simulink model "KINvasion"  (Simulink 7.5)
settings: Solver=ode4  SolverMode=SingleTasking  StartTime=0.0  StopTime=inf  FixedStep=0.0005  RelTol=1e-3
StartFcn:
  |  warndlg('Dexterit-E models cannot run under simulation. Please compile your model and run it from within Dexterit-E.');set_param(gcs,'SimulationCommand','stop')
undefined symbols (not defined in the file or in its folder): Process_Video_CMD, Video
libraries: xpclib x5, General x3, KINARM_general x1, KINARM_EP_loads x1
(part 2 of 3)

== stateflow chart Trial_Control ==
  settings: sampleTime=0.001
  state Initialize/
    // Initialize all variables at the start of the game
    logging_enable = 0;
    game_state=0;
    InitializeAll();
    NullVCODES();
    Continue=1;
  state Main_Trial/
    state GameOn/
      // Set up a level and run the game
      logging_enable=1;
      EnemyNum=Trial_Protocol[EnemyNumber];
      Difficulty=Trial_Protocol[DifficultyNumber];
      MoneyNum=Trial_Protocol[MoneyDrops];
      BossNum=Trial_Protocol[BossNumber];
      GameLoop(1);
      during:
      GameLoop(0);
      exit:
      TitleText();
      ZeroForce();
    state Win/
      // The player won.
      // Continue to interstate
    state Loss/
      // The player lost
      // Set variable to skip
      // all futher levels
      Continue=0;
    state Store/
      // Show the store to the player
      game_state=0;
      ZeroForce();
      Level=Level+1;
      during:
      StoreLoop();
    GameOn -> Win [order 2] : [game_state==2]
    GameOn -> Loss [order 1] : [game_state==3]
    Store -> GameOn : [game_state==1 || TWP[DemoMode]!=0]
  state Inter_Trial_State/
    tickCount=10;
    logging_enable = 0;
    e_Trial_End;
  state Continuing/
    // Does the player get
    // to play another
    // level or did they
    // lose?
  Main_Trial -> Inter_Trial_State : e_ExitTrialNow/
      | // if e_ExitTrialNow event occurs,
      | tickCount=1;
  Initialize -> Store
  (default) -> Initialize
  Win -> Inter_Trial_State : after(2000, e_clk)
  Inter_Trial_State -> Continuing : after(tickCount, e_clk)
  Loss -> Inter_Trial_State : after(10000, e_clk)
  Continuing -> Store [order 1] : [Continue==1]
  Continuing -> Inter_Trial_State [order 2] : [Continue==0]
  data: Initialize function_input double; RRRGGGBBB function_input double; RRGGBBAA function_output uint32; out function_output double size=[1 2]; in function_input double; out function_output double size=[1 3]; in function_input double; logging_enable output double; Trial_Protocol input double; tickCount local double; EnemyNum local double; Difficulty local double; game_state local double; Forces output double size=[1 4]; Continue local double; Money local double; Score local double; VCODES output double size=[100,70]; Upgrades local double size=5; TWP input double; KINARMdata input double; ForcePlatedata input double; seed input double; Level local double; MoneyNum local double; BossNum local double
  events: e_clk input RISING_EDGE_EVENT; e_ExitTrialNow input EITHER_EDGE_EVENT; e_Trial_End output EITHER_EDGE_EVENT
  function StoreLoop:
    | function StoreLoop
    | % This function shows and regulates the game's behaviour while the player
    | % is buying and selling upgrades.
    | %
    | % Upgrades is a 1x5 vector that tracks how many of each upgrade the player
    | % has purchased.
    | %
    | 
    |     persistent SelectTimer; % Used to limit time between purchases
    |     
    |     Forces=zeros(1,4); % Don't need forces here
    |     
    |     if isempty(SelectTimer)
    |         SelectTimer=0;
    |     end
    |     
    |     VCODES=zeros(100,70);
    |     
    |     % increments of vertical space for display
    |     increment=(TWP(WindowMaxY)-TWP(WindowMinY))/8; 
    |     
    |     for i=1:2
    |         if i==1
    |             active_arm=KINARMdata(3,1);			%choose dominant arm first
    |         else
    |             active_arm=3-KINARMdata(3,1);		%choose non-dominant arm 2nd
    |         end
    |         
    |         VCODES(i,1)=1;							%target_type of circle
    |         VCODES(i,2)=1;                          %show target
    |         VCODES(i,5)=colourshift(100255);        %fill colour
    |         VCODES(i,6)=colourshift(100255);		%stroke colour
    |         VCODES(i,7)=0;							%no stroke width
    |         VCODES(i,9)=100;                        %100% opacity
    |         VCODES(i,10)=0.005;                     %radius (m)
    |         feedfwd=KINARMdata(3,2);
    |         VCODES(i,3)=KINARMdata(active_arm,23) + KINARMdata(active_arm,25)*feedfwd;
    |         VCODES(i,4)=KINARMdata(active_arm,24) + KINARMdata(active_arm,26)*feedfwd;
    |         
    |         if SelectTimer==0
    |             % If using the right hand, buy things
    |             if ((sum(KINARMdata(active_arm,47:48).^2)>TWP(FireTorque)^2)&& i==1)
    |                 SelectTimer=600;
    |                 if (IsOver(VCODES(i,4))==2 && Money>=10)
    |                     Money=Money-10;
    |                     Upgrades(1)=Upgrades(1)+1;
    |                 elseif (IsOver(VCODES(i,4))==3 && Money>=15)
    |                     Money=Money-15;
    |                     Upgrades(2)=Upgrades(2)+1;
    |                 elseif (IsOver(VCODES(i,4))==4 && Money>=25)
    |                     Money=Money-25;
    |                     Upgrades(4)=Upgrades(4)+1;
    |                 elseif (IsOver(VCODES(i,4))==5 && Money>=50)
    |                     Money=Money-50;
    |                     Upgrades(3)=Upgrades(3)+1;
    |                 elseif IsOver(VCODES(i,4))==7
    |                     game_state=1;
    |                 end
    |                     
    |             % If using the left hand, sell things
    |             elseif ((sum(KINARMdata(active_arm,47:48).^2)>TWP(FireTorque)^2)&& i==2)
    |                 SelectTimer=600;
    |                 if (IsOver(VCODES(i,4))==2 && Upgrades(1)>=1)
    |                     Money=Money+10;
    |                     Upgrades(1)=Upgrades(1)-1;
    |                 elseif (IsOver(VCODES(i,4))==3 && Upgrades(2)>=1)
    |                     Money=Money+15;
    |                     Upgrades(2)=Upgrades(2)-1;
    |                 elseif (IsOver(VCODES(i,4))==4 && Upgrades(4)>=1)
    |                     Money=Money+25;
    |                     Upgrades(4)=Upgrades(4)-1;
    |                 elseif (IsOver(VCODES(i,4))==5 && Upgrades(3)>=1)
    |                     Money=Money+50;
    |                     Upgrades(3)=Upgrades(3)-1;
    |                 elseif IsOver(VCODES(i,4))==7
    |                     game_state=1;
    |                 end
    |             end
    |         else
    |             SelectTimer=SelectTimer-1;
    |         end
    |         
    |     end
    |     
    |     % Show score and money
    |     VCODES(3,:)=titleCode(...
    |         ['SCORE ',numberText3(Score),' $',numberText3(Money)],...
    |         [TWP(WindowMaxX),TWP(WindowMaxY)],0.05);
    |     
    |     % Show buying options
    |     VCODES(4,:)=titleCode(['Shields          $10 / ',(48+floor(Upgrades(1)/10)), 48+mod(Upgrades(1),10)],...
    |         [(TWP(WindowMaxX)+TWP(WindowMinX))/2,(TWP(WindowMaxY)-increment*2)],0.04);
    |     VCODES(5,:)=titleCode(['Charge Rate     $15 / ',(48+floor(Upgrades(2)/10)), 48+mod(Upgrades(2),10)],...
    |         [(TWP(WindowMaxX)+TWP(WindowMinX))/2,(TWP(WindowMaxY)-increment*3)],0.04);
    |     VCODES(6,:)=titleCode(['Bombs          $25 / ',(48+floor(Upgrades(4)/10)), 48+mod(Upgrades(4),10)],...
    |         [(TWP(WindowMaxX)+TWP(WindowMinX))/2,(TWP(WindowMaxY)-increment*4)],0.04);
    |     VCODES(7,:)=titleCode(['AutoCannon  $50 / ',(48+floor(Upgrades(3)/10)), 48+mod(Upgrades(3),10)],...
    |         [(TWP(WindowMaxX)+TWP(WindowMinX))/2,(TWP(WindowMaxY)-increment*5)],0.04);
    |     
    |     % Show option to continue to the play stage
    |     VCODES(8,:)=titleCode('DONE',...
    |         [(TWP(WindowMaxX)+TWP(WindowMinX))/2,(TWP(WindowMaxY)-increment*7)],0.04);
    | 
    | end
    | 
    | %%%%%%%%%%%%%  ADDITIONAL FUNCTIONS %%%%%%%%%%%%%%%
    | 
    | function VC = titleCode(str,loc,size)
    | % This function creates a VCODE with some text at a certain
    | % size and global location.
    | 
    |     VC=zeros(1,70);
    |     VC(1,1)=11;                             %target_type of labelled circle
    |     VC(1,2)=1;                              %show target
    |     VC(1,3) = loc(1);
    |     VC(1,4) = loc(2);
    |     VC(1,5)=colourshift(255);               %fill colour
    |     VC(1,6)=colourshift(255);               %stroke colour
    |     VC(1,7)=0.00;                           %no stroke width
    |     VC(1,9)=100;                            %100% opacity
    |     VC(1,10)=0.0;                           %radius (m)
    |     VC(1,15:(length(str)+14))=uint16(str);  %str in letters
    |     VC(1,65)=colourshift(254254254);        %text color
    |     VC(1,66)=size;                          %text height (m)
    |     
    | end
    | 
    | function inc=IsOver(locy)
    | % This function finds the increment of vertical space that the location
    | % is in. To allow for discrimination of choices
    | 
    |     inc=TWP(WindowMaxY)-locy;
    |     inc=inc/((TWP(WindowMaxY)-TWP(WindowMinY))/8);
    |     inc=floor(inc+0.5);
    | 
    | end
  function GameLoop(Initialize):
    | function GameLoop(Initialize)
    | % This function is iterated every millisecond of game time. It shows all
    | % the graphics by creating VCODEs, and updates the location and state of
    | % all game elements.
    | 
    |     % Some persistent variables that are needed between game loop iterations
    |     persistent Power Health Shields Enemies Bosses Shots firstrun startcounter forcedata Bombs Moneys;
    |     
    |     MaxShips=50;
    |     MaxShots=70;
    |     MaxMoneys=50;
    |     MaxBosses=15;
    |     
    |     % Instantiate random seed.
    |     if isempty(firstrun)
    |         rand('twister',seed);
    |         firstrun=1;
    |     end
    | 
    |     Forces=zeros(1,4);
    |     T=[0,0];
    |     temp=0;
    |     
    |     VCODES=zeros(100,70);
    |     
    |     if (isempty(forcedata) || Initialize==1)
    |         forcedata=[ForcePlatedata(10),ForcePlatedata(3),0,0];
    |     end
    |     forcedata(3:4)=abs([ForcePlatedata(10),ForcePlatedata(3)]-forcedata(1:2));
    |     forcedata(1:2)=[ForcePlatedata(10),ForcePlatedata(3)];
    |     
    |     if (isempty(Bombs) || Initialize==1)
    |         Bombs=[0,0,0,0,0,0];
    |     end
    |     
    |     
    |     if (isempty(Power) || Initialize==1)
    |         Power=[100,100,100];
    |     end
    |     
    |     if (isempty(Health) || Initialize==1)
    |         Health=0;
    |     end
    |     
    |      if (isempty(Shields) || Initialize==1)
    |         Shields=0;
    |     end
    |     
    |     if (isempty(startcounter) || Initialize==1)
    |         startcounter=1;
    |     end
    |     
    |     if (isempty(Shots) || Initialize==1)
    |         Shots=zeros(MaxShots,6);
    |     end
    |     
    |     if isempty(Enemies)
    |         Enemies=zeros(MaxShips,9);
    |     end
    |     
    |     if isempty(Bosses)
    |         Bosses=zeros(MaxBosses,9);
    |     end
    |     
    |     if isempty(Moneys)
    |         Moneys=zeros(MaxMoneys,3);
    |     end
    |     
    |     % Function to set up enemies, bosses, and money drops at the start of
    |     % each level.
    |     if (Initialize==1)
    |         Enemies=zeros(MaxShips,9);
    |         for i=1:EnemyNum
    |             Enemies(i,:)=[  100,...                 % Health
    |                             30*rand(),...           % Power
    |                             rand()*(TWP(WindowMaxX)-TWP(WindowMinX))+TWP(WindowMinX),...     % X
    |                             (rand()*0.5+0.5+5.0*i/EnemyNum)*(TWP(WindowMaxY)-TWP(WindowMinY))+TWP(WindowMinY),...     % Y
    |                             (rand()*0.02-0.01)*Difficulty,...       % dX
    |                             0,...                                   % dY
    |                             0,...                                   % ddX
    |                             0,...                                   % ddY
    |                             rand()*50+10];                          % frequency
    |         end
    |         
    |         Bosses=zeros(MaxBosses,9);
    |         for i=1:BossNum
    |             Bosses(i,:)=[   200*Difficulty+500+500*i,...  % Health
    |                             floor(1000*rand()),...        % WeaponCounter
    |                             rand()*(TWP(WindowMaxX)-TWP(WindowMinX))+TWP(WindowMinX),...     % X
    |                             (1+1.0*i/BossNum)*(TWP(WindowMaxY)-TWP(WindowMinY))+TWP(WindowMinY),...     % Y
    |                             (rand()*0.02-0.01)*Difficulty,...     % dX
    |                             0,...                                 % dY
    |                             0,...                                 % ddX
    |                             0,...                                 % ddY
    |                             0];                                   % unused
    |         end
    |         
    |         Moneys=zeros(MaxMoneys,3);
    |         for i=1:MoneyNum
    |             Moneys(i,:)=[  max(1,floor((rand()+rand())*3-2)),...  % money in this drop
    |                            rand()*(TWP(WindowMaxX)-TWP(WindowMinX))+TWP(WindowMinX),...  % X
    |                            (rand()*0.5+0.5+10.0*i/MoneyNum)*(TWP(WindowMaxY)-TWP(WindowMinY))+TWP(WindowMinY)]; % Y
    |         end
    |                            
    |     end
    |     
    | 
    |     %Setup Ship Vcodes
    |     for i=1:2
    |         
    |         % Show a circle at each hand whose radius shows power level.
    |         if i==1
    |             active_arm=KINARMdata(3,1);			%choose dominant arm first
    |         else
    |             active_arm=3-KINARMdata(3,1);		%choose non-dominant arm 2nd
    |         end
    |         T(i)=sqrt(KINARMdata(active_arm,47)^2+KINARMdata(active_arm,48)^2);
    |         VCODES(i,1)=1;							%target_type of circle
    |         VCODES(i,2)=1;                          %show target
    |         VCODES(i,5)=colourshift(255);			%fill colour
    |         VCODES(i,6)=colourshift(255);			%stroke colour
    |         VCODES(i,7)=0;							%no stroke width
    |         VCODES(i,9)=100;                        %100% opacity
    |         VCODES(i,10)=0.00015*Power(i);          %radius (m)
    |         feedfwd=KINARMdata(3,2);
    |         VCODES(i,3)=KINARMdata(active_arm,23) + KINARMdata(active_arm,25)*feedfwd;
    |         VCODES(i,4)=KINARMdata(active_arm,24) + KINARMdata(active_arm,26)*feedfwd;
    |         
    |     end
    |     
    |     % Show a bar between the hands that represents health.
    |     VCODES(3,1)=4;						%target_type of line
    |     VCODES(3,2)=1;                      %show target
    |     VCODES(3,5)=-4;                     %fill colour
    |     VCODES(3,6)=-4;                     %stroke colour
    |     VCODES(3,7)=0.00025*Health;         %stroke width
    |     VCODES(3,9)=100;                    %100% opacity
    |     VCODES(3,3) = VCODES(1,3);          %one end X
    |     VCODES(3,4) = VCODES(1,4);          %one end Y
    |     VCODES(3,10) = VCODES(2,3)-VCODES(1,3); % X vector to other end
    |     VCODES(3,11) = VCODES(2,4)-VCODES(1,4); % Y vector to other end
    |     
    |     % Show the score and money
    |     VCODES(4,:)=titleCode(...
    |         ['SCORE ',numberText3(Score),' $',numberText3(Money)],...
    |         [TWP(WindowMaxX),TWP(WindowMaxY)],0.04);
    |     
    |     C=4;
    |     
    |     % If the player has a shield, show it as an elipse between the hands
    |     if ((Shields>0) && (VCODES(3,10)^2+VCODES(3,11)^2)<0.1)
    |         C=C+1;
    |         VCODES(C,1)=2;                              %target_type of elipse
    |         VCODES(C,2)=1;                              %show target
    |         VCODES(C,5)=colourshift(255);               %fill colour
    |         VCODES(C,6)=colourshift(255);               %stroke colour
    |         VCODES(C,7)=0;                              %no stroke width
    |         VCODES(C,9)=max(min(Shields*0.5,70),10);    %opacity is strength
    |         VCODES(C,3) = VCODES(1,3)+VCODES(3,10)/2;
    |         VCODES(C,4) = VCODES(1,4)+VCODES(3,11)/2;
    |         VCODES(C,10) = sqrt(VCODES(3,10)^2+VCODES(3,11)^2)/2+0.02;
    |         VCODES(C,11) = 0.03;
    |         VCODES(C,12) = atan2(VCODES(3,11),VCODES(3,10));
    |     end
    |     
    |     % If the player has an autocannon, show it as a circle between the hands
    |     if (Upgrades(3)>0)
    |         C=C+1;
    |         VCODES(C,1)=1;							%target_type of circle
    |         VCODES(C,2)=1;                          %show target
    |         VCODES(C,5)=colourshift(255);           %fill colour
    |         VCODES(C,6)=colourshift(200200000);		%stroke colour
    |         VCODES(C,7)=0.003;                      %stroke width
    |         VCODES(C,9)=100;                        %100% opacity
    |         VCODES(C,10)=0.010;                     %radius (m)
    |         VCODES(C,3)=VCODES(1,3)+VCODES(3,10)/2;
    |         VCODES(C,4)=VCODES(1,4)+VCODES(3,11)/2;
    |         
    |     end
    |     
    |     % If the player has bombs, list them at the top of the screen
    |     if (Upgrades(4)>0)
    |         C=C+1;
    |         VCODES(C,:)=titleCode('B ',[TWP(WindowMinX),TWP(WindowMaxY)],0.05);
    |         for i=1:min(Upgrades(4),10)
    |             VCODES(C,16+i)=48;
    |         end
    |     end
    |     
    |     % If within 3000ms of start, show the life bar and shields grow, do not process
    |     % any game updates afterwards. Show a title with the level.
    |     if (startcounter < 3000)
    |         C=C+1;
    |         VCODES(C,:)=titleCode(['LEVEL ',(48+floor(Level/10)),48+mod(Level,10)],[(TWP(WindowMaxX)+TWP(WindowMinX))/2,(TWP(WindowMaxY)+TWP(WindowMinY))/2],0.05);
    |         startcounter=startcounter+1;
    |         Health=min(Health+0.05,100);
    |         
    |         if (startcounter<Upgrades(1)*150)
    |             Shields=Shields+0.07;
    |         end
    |         
    |         return;
    |     end
    |     
    |     % Check for manipulator torque and if power level is high enough, fire
    |     % a shot perpendicular to life bar.
    |     for i=1:2
    |         if Power(i)>25
    |             if T(i)>TWP(FireTorque)
    |                 F=firstzero(Shots(:,1));
    |                 if (F>0)
    |                     
    |                     fv=fireVector([VCODES(1,3)-VCODES(2,3),VCODES(1,4)-VCODES(2,4)]);
    |                     Shots(F,1)=Power(i);
    |                     Shots(F,2)=VCODES(i,3)+fv(1)*0.04;
    |                     Shots(F,3)=VCODES(i,4)+fv(2)*0.04;
    |                     Shots(F,4)=fv(1)*0.3;
    |                     Shots(F,5)=fv(2)*0.3;
    |                     Shots(F,6)=1;
    |                     Power(i)=0;
    |                 end
    |             end
    |         end
    |     end
    |     
    |     % Add more power each loop, as given by Upgrade(2)
    |     temp=sqrt(sum(VCODES(3,10:11).^2));
    |     Power(1)=min(Power(1)+temp*0.1*(Upgrades(2)+5)/5,100);
    |     Power(2)=min(Power(2)+temp*0.1*(Upgrades(2)+5)/5,100);
    |     Power(3)=min(Power(3)+temp*0.1,100);
    |     
    |     % Check for change in forceplate pressure for bomb use
    |     for i=1:2
    |         if (Bombs(i*3)==0 && Upgrades(4)>0)
    |             if (forcedata(2+i)>TWP(StompForce))
    |                 if TWP(DemoMode)==0
    |                     Upgrades(4)=Upgrades(4)-1;
    |                 end
    |                 Bombs(3*i-2)=VCODES(i,3);
    |                 Bombs(3*i-1)=VCODES(i,4);
    |                 Bombs(3*i)=1;
    |             end
    |         end
    |     end
    |     
    |     
    |     % Check through all shots to see if any are within the shields or the
    |     % life bar. If they are, cause damage to the player accordingly.
    |     for j=1:size(Shots,1)
    |         if (Shots(j,1)>0 && Shots(j,6)==0)
    |             if (Shields>0 && (VCODES(3,10)^2+VCODES(3,11)^2)<0.1 && isInsideLine(  Shots(j,2:3) , VCODES(3,[3,4,10,11]) , 0.04  ))
    |                 temp=min(Shields,Shots(j,1));
    |                 Shields=max(0,Shields-temp);
    |                 Shots(j,1)=max(Shots(j,1)-temp,0);
    |             end
    |                 
    |             if isInsideLine(  Shots(j,2:3) , VCODES(3,[3,4,10,11]) , VCODES(3,7)  )
    |                 Health= max(Health-Shots(j,1),0);
    |                 Forces=Forces+[Shots(j,4:5),Shots(j,4:5)]/sqrt(sum(Shots(j,4:5).^2))*Shots(j,1)*0.01*TWP(ForceSize);
    |                 % DO FORCE OUTPUT HERE
    |                 Shots(j,1)=0;
    |             end
    |         end
    |     end
    |     
    |     % Update each money drop, show its VCODE and check to see if the player
    |     % is over it for collection.
    |     for i=1:MaxMoneys
    |         
    |         Moneys(i,3)=Moneys(i,3)-0.0001;
    |         
    |         if Moneys(i,1)<=0
    |             continue;
    |         end
    |         
    |         if ((Moneys(i,3)>TWP(WindowMaxY)) || (Moneys(i,3)<TWP(WindowMinY)))
    |             continue;
    |         end
    |         
    |         C=C+1;
    |         
    |         VCODES(C,1)=11;							%target_type of circle
    |         VCODES(C,2)=1;                          %show target
    |         VCODES(C,3)=Moneys(i,2);           % X
    |         VCODES(C,4)=Moneys(i,3);           % Y
    |         VCODES(C,5)=colourshift(253253000);		%fill colour as specified by GUI
    |         VCODES(C,6)=colourshift(200128000);		%stroke colour same as fill colour
    |         VCODES(C,7)=0.002;						%no stroke width
    |         VCODES(C,9)=100;                    %100% opacity
    |         VCODES(C,10)=(0.005+Moneys(i,1)*0.003);                  %radius (m)
    |         for j=1:Moneys(i,1)
    |             VCODES(C,14+j)=36;
    |         end
    |         VCODES(C,65)=colourshift(200128000);
    |         VCODES(C,66)=0.01;
    |         
    |         if isInsideLine(  Moneys(i,2:3) , VCODES(3,[3,4,10,11]) , VCODES(3,7)  )
    |                 Money=Money+Moneys(i,1);
    |                 Moneys(i,1)=0;
    |         end
    |         
    |     end
    |     
    |     
    |     
    |     wincondition=1; % Used for ending the level if everything is dead
    |     closestloc=[0,0]; % Used for autocannon targetting
    |     closestrange=1000; % Used for autocannon targetting
    |     bossactive=0; % variable to track if a boss is onscreen
    | 
    |     %% UPDATE EACH BOSS %%
    |     for i=1:MaxBosses
    |         
    |         % Move the bosses
    |         if (Bosses(i,4)>(TWP(WindowMinY)+(TWP(WindowMaxY)-TWP(WindowMinY))*(2+bossactive)/(3+bossactive)))
    |             if (Bosses(i,4)>(TWP(WindowMaxY)) && bossactive )
    |                 Bosses(i,4)=Bosses(i,4)-0.000002;
    |             else
    |                 Bosses(i,4)=Bosses(i,4)-0.00001;
    |             end
    |         end
    |         
    |         Bosses(i,3:4)=Bosses(i,3:4)+Bosses(i,5:6)/1000;
    |         
    |         if ((Bosses(i,3)>TWP(WindowMaxX)) && Bosses(i,5)>0)
    |             Bosses(i,5)=-Bosses(i,5);
    |         elseif ((Bosses(i,3)<TWP(WindowMinX)) && Bosses(i,5)<0)
    |             Bosses(i,5)=-Bosses(i,5);
    |         end
    |         
    |         
    |         if Bosses(i,1)<=0
    |             continue;
    |         else
    |             wincondition=0;
    |         end
    |         
    |         if ((Bosses(i,4)>TWP(WindowMaxY)) || (Bosses(i,4)<TWP(WindowMinY)))
    |             continue;
    |         end
    |         
    |         % Check if boss is closest target for autocannon
    |         temp=sum((Bosses(i,3:4)-[VCODES(1,3)+VCODES(3,10)/2,VCODES(1,4)+VCODES(3,11)/2]).^2);
    |         if (temp<closestrange)
    |             closestloc=Bosses(i,3:4);
    |             closestrange=temp;
    |         end
    |         
    |         bossactive=bossactive+1;
    |         
    |         C=C+1;
    |         
    |         VCODES(C,1)=3;							%target_type of line
    |         VCODES(C,2)=1;                          %show target
    |         VCODES(C,3)=Bosses(i,3);           % X
    |         VCODES(C,4)=Bosses(i,4);           % Y
    |         VCODES(C,5)=-5;		%fill colour as specified by GUI
    |         VCODES(C,6)=-5;		%stroke colour same as fill colour
    |         VCODES(C,7)=0;						%no stroke width
    |         VCODES(C,9)=Bosses(i,1)*0.1+50;                    %100% opacity
    |         VCODES(C,10)=0.20;                  %radius (m)
    |         VCODES(C,11)=0.07;                  %radius (m)
    |         
    |         % See if the boss is hit by any shots
    |         for j=1:MaxShots
    |             if (Shots(j,1)>0 && Shots(j,6)==1 && isInsideLine(Shots(j,2:3),[Bosses(i,3)-VCODES(C,10)/2,Bosses(i,4),VCODES(C,10),0.0],VCODES(C,11)))
    |                 Bosses(i,1)= max(Bosses(i,1)-Shots(j,1),0);
    |                 Bosses(i,5:6)= Bosses(i,5:6)+Shots(j,4:5)*0.0; %impact force
    |                 Shots(j,1)=0;
    |             end
    |         end
    |         
    |         % See if the boss is within the radius of any exploding bombs
    |         if (Bombs(3)>0 && isInsideCircle(Bosses(i,3:4),Bombs(1:2),Bombs(3)/1000))
    |             Bosses(i,1)= max(Bosses(i,1)-1,0);
    |         end
    |         if (Bombs(6)>0 && isInsideCircle(Bosses(i,3:4),Bombs(4:5),Bombs(6)/1000))
    |             Bosses(i,1)= max(Bosses(i,1)-1,0);
    |         end
    |             
    |         % See if the boss is within the shields or lifebar of the player (collision)
    |         if (Shields>0 && (VCODES(3,10)^2+VCODES(3,11)^2)<0.1 && isInsideLine(  Bosses(i,3:4) , VCODES(3,[3,4,10,11]) , 0.04  ))
    |             temp=min(Shields,Bosses(i,1)*0.5);
    |             Shields=max(0,Shields-temp);
    |             Bosses(i,1)=max(Bosses(i,1)-temp*2,0);
    |         end
    |         
    |         if (isInsideLine(  Bosses(i,3:4) , VCODES(3,[3,4,10,11]) , VCODES(3,7)  ))
    |             Health= max(Health-Bosses(i,1)*0.5,0);
    |             Forces=Forces+[0,-TWP(ForceSize)*min(Bosses(i,1),100)*0.01,0,-TWP(ForceSize)*min(Bosses(i,1),100)*0.01];
    |             Bosses(i,1)=0;
    |         end
    |         
    |         % Check the bosses timer and apply various weaponry
    |         if mod(Bosses(i,2),2000/Difficulty)==0
    |             F=firstzero(Shots(:,1));
    |             if (F>0)
    |                 temploc=[Bosses(i,3)+VCODES(C,10)/2*(rand()-0.5),Bosses(i,4)];
    |                 v=vectorTo(temploc,(VCODES(3,3:4)+VCODES(3,10:11)./2),(1/(Difficulty*1.5)));
    |                 Shots(F,1)=9+Difficulty*2;
    |                 Shots(F,2)=temploc(1)+v(1)*(0.021+0.02/Difficulty);
    |                 Shots(F,3)=temploc(2)+v(2)*(0.021+0.02/Difficulty);
    |                 Shots(F,4)=v(1)*(0.03*Difficulty+0.07);
    |                 Shots(F,5)=v(2)*(0.03*Difficulty+0.07);
    |                 Shots(F,6)=0;
    |             end
    |         end
    |         
    |         if mod(Bosses(i,2),10000/Difficulty)==0
    |             F=firstzero(Shots(:,1));
    |             if (F>0)
    |                 v=vectorTo(Bosses(i,3:4),(VCODES(3,3:4)+VCODES(3,10:11)./2),(1/(Difficulty*1.5)));
    |                 Shots(F,1)=100;
    |                 Shots(F,2)=Bosses(i,3)+v(1)*(0.021+0.02/Difficulty);
    |                 Shots(F,3)=Bosses(i,4)+v(2)*(0.021+0.02/Difficulty);
    |                 Shots(F,4)=v(1)*(0.01*Difficulty+0.04);
    |                 Shots(F,5)=v(2)*(0.01*Difficulty+0.04);
    |                 Shots(F,6)=0;
    |             end
    |         end
    |         
    |         if mod(Bosses(i,2),30000/Difficulty)==0
    |             for j=1:12
    |                 angle=j/6*3.1415;
    |                 F=firstzero(Shots(:,1));
    |                 if (F>0)
    |                     v=[cos(angle),sin(angle)];
    |                     Shots(F,1)=50;
    |                     Shots(F,2)=Bosses(i,3)+v(1)*(0.021+0.02/Difficulty);
    |                     Shots(F,3)=Bosses(i,4)+v(2)*(0.021+0.02/Difficulty);
    |                     Shots(F,4)=v(1)*(0.01*Difficulty+0.04);
    |                     Shots(F,5)=v(2)*(0.01*Difficulty+0.04);
    |                     Shots(F,6)=0;
    |                 end
    |             end
    |         end
    |         
    |         Bosses(i,2)=mod(Bosses(i,2)+1,30001);
    |         
    |         % If the boss is dead, add some score and money to the player
    |         if Bosses(i,1)==0
    |             Money=Money+TWP(MoneyPerShip)*5;
    |             Score=Score+5;
    |         end
    |         
    |     end
    |     
    |     %% UPDATE EACH ENEMY %%
    |     for i=1:MaxShips
    |         
    |         % Move the enemy
    |         if (bossactive==0 || Enemies(i,4)<TWP(WindowMaxY))
    |             Enemies(i,4)=Enemies(i,4)-0.00005;
    |         else
    |             Enemies(i,4)=Enemies(i,4)-0.00001;
    |         end
    |         
    |         if ((Enemies(i,3)>TWP(WindowMaxX)) && Enemies(i,5)>0)
    |             Enemies(i,5)=-Enemies(i,5);
    |         elseif ((Enemies(i,3)<TWP(WindowMinX)) && Enemies(i,5)<0)
    |             Enemies(i,5)=-Enemies(i,5);
    |         end
    |         
    |         if Enemies(i,1)<=0
    |             continue;
    |         end
    |         
    |         if (Enemies(i,4)>TWP(WindowMinY))
    |             wincondition=0;
    |         end
    |         
    |         if ((Enemies(i,4)>TWP(WindowMaxY)) || (Enemies(i,4)<TWP(WindowMinY)))
    |             continue;
    |         end
    |         
    |         % Check if enemy is closest target for autocannon
    |         temp=sum((Enemies(i,3:4)-[VCODES(1,3)+VCODES(3,10)/2,VCODES(1,4)+VCODES(3,11)/2]).^2);
    |         if (temp<closestrange)
    |             closestloc=Enemies(i,3:4);
    |             closestrange=temp;
    |         end
    |         
    |         C=C+1;
    |         
    |         VCODES(C,1)=1;							%target_type of circle
    |         VCODES(C,2)=1;                          %show target
    |         VCODES(C,3)=Enemies(i,3);           % X
    |         VCODES(C,4)=Enemies(i,4);           % Y
    |         VCODES(C,5)=-1;		%fill colour as specified by GUI
    |         VCODES(C,6)=-1;		%stroke colour same as fill colour
    |         VCODES(C,7)=0;						%no stroke width
    |         VCODES(C,9)=Enemies(i,1)*0.5+50;                    %100% opacity
    |         VCODES(C,10)=0.02+0.02*(Enemies(i,2)*0.01);                  %radius (m)
    |         
    |         % See if the enemy is hit by any shots
    |         for j=1:MaxShots
    |             if (Shots(j,1)>0 && Shots(j,6)==1 && isInsideCircle(Shots(j,2:3),Enemies(i,3:4),(0.02/Difficulty)+0.01))
    |                 Enemies(i,1)= max(Enemies(i,1)-Shots(j,1),0);
    |                 Enemies(i,5:6)= Enemies(i,5:6)+Shots(j,4:5)*0.0; %impact force
    |                 Shots(j,1)=0;
    |             end
    |         end
    |         
    |         % See if the enemy is within the radius of any exploding bombs
    |         if (Bombs(3)>0 && isInsideCircle(Enemies(i,3:4),Bombs(1:2),Bombs(3)/1000))
    |             Enemies(i,1)= max(Enemies(i,1)-1,0);
    |         end
    |         if (Bombs(6)>0 && isInsideCircle(Enemies(i,3:4),Bombs(4:5),Bombs(6)/1000))
    |             Enemies(i,1)= max(Enemies(i,1)-1,0);
    |         end
    |             
    |         % See if the enemy is within the shields or lifebar of the player (collision)
    |         if (Shields>0 && (VCODES(3,10)^2+VCODES(3,11)^2)<0.1 && isInsideLine(  Enemies(i,3:4) , VCODES(3,[3,4,10,11]) , 0.04  ))
    |             temp=min(Shields,Enemies(i,1)*0.5);
    |             Shields=max(0,Shields-temp);
    |             Enemies(i,1)=max(Enemies(i,1)-temp*2,0);
    |         end
    |         
    |         if (isInsideLine(  Enemies(i,3:4) , VCODES(3,[3,4,10,11]) , VCODES(3,7)  ))
    |             Health= max(Health-Enemies(i,1)*0.5,0);
    |             Forces=Forces+[0,-TWP(ForceSize)*Enemies(i,1)*0.01,0,-TWP(ForceSize)*Enemies(i,1)*0.01];
    |             Enemies(i,1)=0;
    |         end
    |         
    |         % Check to see if the enemy's power level is high enough, an fire a shot
    |         if Enemies(i,2)>Enemies(i,9)
    |             F=firstzero(Shots(:,1));
    |             if (F>0)
    |                 v=vectorTo(Enemies(i,3:4),(VCODES(3,3:4)+VCODES(3,10:11)./2),(1/(Difficulty*1.5)));
    |                 Shots(F,1)=Enemies(i,2);
    |                 Shots(F,2)=Enemies(i,3)+v(1)*(0.021+0.02/Difficulty);
    |                 Shots(F,3)=Enemies(i,4)+v(2)*(0.021+0.02/Difficulty);
    |                 Shots(F,4)=v(1)*(0.03*Difficulty+0.07);
    |                 Shots(F,5)=v(2)*(0.03*Difficulty+0.07);
    |                 Shots(F,6)=0;
    |                 Enemies(i,2)=0;
    |             end
    |         end
    |         
    |         % regen some power
    |         Enemies(i,2)=Enemies(i,2)+TWP(BaseRegen)*0.001*(Difficulty+2)/3;
    |         
    |          % If the enemy is dead, add some score and money to the player
    |         if Enemies(i,1)==0
    |             Money=Money+TWP(MoneyPerShip);
    |             Score=Score+1;
    |         end
    | 
    |     end
    |     
    |     
    |     
    |     % AutoCannon firing if we have a target
    |     if (Upgrades(3)>0 && closestrange<1000)
    |         if (Power(3)>=25)
    |             F=firstzero(Shots(:,1));
    |             if (F>0)
    |                 fv=autoVector([VCODES(1,3)+VCODES(3,10)/2,VCODES(1,4)+VCODES(3,11)/2],closestloc);
    |                 Shots(F,1)=Upgrades(3)*20;
    |                 Shots(F,2)=VCODES(1,3)+VCODES(3,10)/2+fv(1)*0.04;
    |                 Shots(F,3)=VCODES(1,4)+VCODES(3,11)/2+fv(2)*0.04;
    |                 Shots(F,4)=fv(1)*0.3;
    |                 Shots(F,5)=fv(2)*0.3;
    |                 Shots(F,6)=1;
    |                 Power(3)=0;
    |             end
    |         end
    |     end
    |     
    |     % If either hand's bomb is active, show it and update its radius
    |     for i=1:2
    |         if Bombs(3*i)>0
    |             Bombs(3*i)=Bombs(3*i)+1;
    |             C=C+1;
    |             VCODES(C,1)=1;							%target_type of circle
    |             VCODES(C,2)=1;                          %show target
    |             VCODES(C,3)=Bombs(3*i-2);           % X
    |             VCODES(C,4)=Bombs(3*i-1);           % Y
    |             VCODES(C,5)=colourshift(255255000);		%fill colour as specified by GUI
    |             VCODES(C,6)=colourshift(255255000);		%stroke colour same as fill colour
    |             VCODES(C,7)=0;						%no stroke width
    |             VCODES(C,9)=70-Bombs(3*i)/10;                    %100% opacity
    |             VCODES(C,10)=Bombs(3*i)/1000;                  %radius (m)
    |             
    |             if Bombs(3*i)>TWP(BombSize)
    |                 Bombs(3*i)=0;
    |             end
    |         end
    |     end
    |     
    |     % Update the trajectory of each shot
    |     for j=1:MaxShots
    |         if Shots(j,1)>0
    |             C=C+1;
    |             VCODES(C,1)=3;							%target_type of circle
    |             VCODES(C,2)=1;                          %show target
    |             VCODES(C,3)=Shots(j,2);           % X
    |             VCODES(C,4)=Shots(j,3);           % Y
    |             VCODES(C,5)=-3+Shots(j,6);		%fill colour as specified by GUI
    |             VCODES(C,6)=-3+Shots(j,6);		%stroke colour same as fill colour
    |             VCODES(C,7)=0;						%no stroke width
    |             VCODES(C,9)=100;                    %100% opacity
    |             VCODES(C,10)=(0.004+0.00005*Shots(j,1))*4;                  %radius (m)
    |             VCODES(C,11)=0.004+0.00005*Shots(j,1);
    |             VCODES(C,12)=atan2(Shots(j,5),Shots(j,4));
    |             
    |             % If the shot is offscreen, delete it
    |             Shots(j,2:3)=Shots(j,2:3)+Shots(j,4:5)*0.001;
    |             if (...
    |                        Shots(j,2)<(TWP(WindowMinX)-0.1)...
    |                     || Shots(j,2)>(TWP(WindowMaxX)+0.1)...
    |                     || Shots(j,3)<(TWP(WindowMinY)-0.1)...
    |                     || Shots(j,3)>(TWP(WindowMaxY)+0.1))
    |                 Shots(j,1)=0;
    |             end
    |             
    |             % If the shot is within a bomb, degrade it.
    |             if (Bombs(3)>0 && isInsideCircle(Bombs(1:2),Shots(j,2:3),Bombs(3)/1000))
    |                 Shots(j,1)= max(Shots(j,1)-1,0);
    |             end
    |             if (Bombs(6)>0 && isInsideCircle(Bombs(4:5),Shots(j,2:3),Bombs(6)/1000))
    |                 Shots(j,1)= max(Shots(j,1)-1,0);
    |             end
    |             
    |         end
    |     end
    |     
    |     % If the player's health is zero, lose.
    |     % If everything is dead or passed, win.
    |     if Health<=0
    |             game_state=3;
    |     elseif (((sum(Enemies(:,1))<1) && (sum(Bosses(:,1))<1)) || wincondition)
    |             game_state=2;
    |     end
    |         
    | end
    | 
    | 
    | %%%%%%%% IN TARGET CALCULATIONS %%%%%%%%%%%
    | 
    | function intarget = isInsideCircle(pos,Cpos,Crad)
    |     delta=pos-Cpos;
    | 	intarget = ((delta(1)^2 + delta(2)^2) <= Crad.^2);
    | end
    | 
    | function v = vectorTo(pos,pos2,err)
    |     v=pos2-pos+rand(1,2)*err-err/2;
    |     v=v./sqrt(v(1)^2+v(2)^2);
    | end
    | 
    | function v = fireVector(pos)
    |     v=[-pos(2),pos(1)];
    |     v=v./sqrt(v(1)^2+v(2)^2);
    | end
    | 
    | function v = autoVector(pos,pos2)
    |     v=pos2-pos;
    |     offset=sqrt(sum(v.^2))/0.3*0.05;
    |     v=v-[0,offset];
    |     v=v./sqrt(v(1)^2+v(2)^2);
    | end
    | 
    | 
    | function intarget = isInsideLine( pos, Lpos, height1 )
    |     
    |     delta=pos-Lpos(1:2);
    |     
    |     w = sqrt(Lpos(3)^2 + Lpos(4)^2);                          %width (cm)
    |     
    |     % determine the vector from the line's midpoint to the hand position
    |     handx = delta(1) - Lpos(3)/2;
    |     handy = delta(2) - Lpos(4)/2;
    |     
    |     t = atan2(Lpos(4), Lpos(3));                                %calculate angle of the line (rads)
    |     sint = sin(t);
    |     cost = cos(t);
    |     
    |     xrotate = handx.*cost + handy.*sint;   %location of x point in rectangle's coordinate frame
    |     yrotate = -handx.*sint + handy.*cost;  %location of y point in rectangle's coordinate frame
    |     
    |     intarget = abs(xrotate) <= w/2 & abs(yrotate) <= max(height1,0.001)/2;
    |     
    | 
    | end
    | 
    | 
    | %%%%%%%%%%%%%%%%% ADDITIONAL FUNCTIONS %%%%%%%%%%%%%%%%%%%
    | 
    | function VC = titleCode(str,loc,size)
    | % This function creates a VCODE with some text at a certain
    | % size and global location.
    | 
    |     VC=zeros(1,70);
    |     VC(1,1)=11;                             %target_type of labelled circle
    |     VC(1,2)=1;                              %show target
    |     VC(1,3) = loc(1);
    |     VC(1,4) = loc(2);
    |     VC(1,5)=colourshift(255);               %fill colour
    |     VC(1,6)=colourshift(255);               %stroke colour
    |     VC(1,7)=0.00;                           %no stroke width
    |     VC(1,9)=100;                            %100% opacity
    |     VC(1,10)=0.0;                           %radius (m)
    |     VC(1,15:(length(str)+14))=uint16(str);  %str in letters
    |     VC(1,65)=colourshift(254254254);        %text color
    |     VC(1,66)=size;                          %text height (m)
    |     
    | end
    | 
    | function ret=firstzero(vector)
    |     ret=0;
    |     for i=1:length(vector)
    |         if vector(i)==0
    |             ret=i;
    |             return;
    |         end
    |     end
    | end
    | 
    | % The colourshift function converts an "RRRGGGBBB" colour value to RRGBB (as an uint32).
    | function RRGGBBAA = colourshift(RRRGGGBBB)
    | 
    | blue = cast(mod(RRRGGGBBB, 1000), 'uint32');
    | green = cast(mod(RRRGGGBBB - blue, 1000000) / 1000, 'uint32');
    | red = cast((RRRGGGBBB - (green * 1000) - blue) / 1000000, 'uint32');
    | 
    | RRGGBBAA = bitshift(red, 16) + bitshift(green, 8) + blue;
    | end
    | %%%%%%%%%%%%%%%%%%%%%%%%%%%%%%%%%%%%%%%%%%%
    | 
    | 
    | 
    |     
    | % VCODEs are length 70. All units in a VCODE should be SI, e.g. (m) and (rad). Elements in a VCODE are defined as follows:
    | %
    | % For all target types:
    | %  1: target type
    | %       1 - circle
    | %       2 - ellipse
    | %       3 - rectangle
    | %       4 - line
    | %       5 - triangle
    | %       11 - circle with label
    | %       12 - ellipse with label
    | %       13 - rectangle with label
    | %       14 - line with label
    | %       15 - triangle with label
    | %  2: target on/off status and target display (which display target will appear on)
    | %		0 - off
    | %		1 - on, appearing on both subject and operator displays
    | %       2 - on, appearing on subject display only
    | %       3 - on, appearing on operator display only
    | %  3: x position (m)
    | %  4: y position (m)
    | %  5: fill colour (RRGGBB) or texture index
    | %  6: stroke colour (RRGGBB) or texture index
    | %  7: stroke width
    | %  8: reserved for target background ID
    | %  9: opacity
    | %
    | % For circles:
    | %  10: radius (m)
    | %
    | % For ellipses:
    | %  10: major radius (m)
    | %  11: minor radius (m)
    | %  12: orientation of major axis (rad)
    | %
    | % For rectangles:
    | %  10: length (m)
    | %  11: height (m)
    | %  12: orientation (rad) (relative to x, y already shown)
    | %
    | % For lines:
    | %  10: endpoint x-axis coordinate relative to start point (m)
    | %  11: endpoint y-axis coordinate relative to start point (m)
    | %
    | % For triangles:
    | %  10: length (m)
    | %  11: height (m)
    | %  12: offset of peak from midpoint of length (m)
    | %  13: orientation (rad)
    | %
    | % For all labelled target types:
    | %  14: reserved
    | %  15-64: label characters (indexes in ISO 8859-1 character set)
    | %  65: label colour (0xRRGBBAA)
    | %  66: label height (m)
    | %  67: reserved
    | %  68: reserved
    | %  69: reserved
    | %  70: reserved
  function TitleText:
    | function TitleText
    | % This function simply shows title text in the center of the screen
    | 
    |     Forces=zeros(1,4);
    |     T=[0,0];
    |     
    |     VCODES=zeros(100,70);
    | 
    |     locx=(TWP(WindowMaxX)+TWP(WindowMinX))/2;
    |     locy=(TWP(WindowMaxY)+TWP(WindowMinY))/2;
    |     
    |     if game_state==2
    |         VCODES(1,:)=titleCode('LEVEL COMPLETE',[locx,locy],0.05);
    |     elseif game_state==3
    |         VCODES(1,:)=titleCode('GAME OVER',[locx,locy*1.3],0.05);
    |         VCODES(2,:)=titleCode('FINAL SCORE',[locx,locy],0.05);
    |         VCODES(3,:)=titleCode(numberText3(Score),[locx,locy*0.7],0.05);
    |     else
    |         VCODES(1,:)=titleCode('READY',[locx,locy],0.05);
    |     end
    |     
    | end
    | 
    | %%%%%%%%%% ADDITIONAL FUNCTIONS %%%%%%%%%%%%%
    | 
    | function VC = titleCode(str,loc,size)
    | % This function creates a VCODE with some text at a certain
    | % size and global location.
    | 
    |     VC=zeros(1,70);
    |     VC(1,1)=11;                             %target_type of labelled circle
    |     VC(1,2)=1;                              %show target
    |     VC(1,3) = loc(1);
    |     VC(1,4) = loc(2);
    |     VC(1,5)=colourshift(255);               %fill colour
    |     VC(1,6)=colourshift(255);               %stroke colour
    |     VC(1,7)=0.00;                           %no stroke width
    |     VC(1,9)=100;                            %100% opacity
    |     VC(1,10)=0.0;                           %radius (m)
    |     VC(1,15:(length(str)+14))=uint16(str);  %str in letters
    |     VC(1,65)=colourshift(254254254);        %text color
    |     VC(1,66)=size;                          %text height (m)
    |     
    | end
  function NullVCODES:
    | function NullVCODES
    |   
    |     VCODES=zeros(100,70);
    | 
    | end
  function InitializeAll:
    | function InitializeAll
    |   
    |     Level=0;
    |    
    |     Money=TWP(StartingMoney);
    |     Score=0;
    |     if TWP(DemoMode)==0
    |         Upgrades=[0;0;0;0;0];
    |     else 
    |         Upgrades=[5;10;1;5;0];
    |     end
    |     Forces=[0 0 0 0];
    | 
    | end
  function ZeroForce:
    | function ZeroForce
    |   
    |     Forces=[0 0 0 0];
    | 
    | end
  function RRGGBBAA = colourshift(RRRGGGBBB):
    | function RRGGBBAA = colourshift(RRRGGGBBB)
    | % This function takes an RGB color and transforms it into VCODE
    | % color values.
    |     blue = cast(mod(RRRGGGBBB, 1000), 'uint32');
    |     green = cast(mod(RRRGGGBBB - blue, 1000000) / 1000, 'uint32');
    |     red = cast((RRRGGGBBB - (green * 1000) - blue) / 1000000, 'uint32');
    | 
    |     RRGGBBAA = bitshift(red, 16) + bitshift(green, 8) + blue;
    | end
  function out=numberText2(in):
    | function out=numberText2(in)
    | % This function takes a number (in) and converts it to
    | % a two-digit character output. Useful for VCODES.
    |     o=floor(mod(in,10));
    |     t=floor(mod(in,100)/10);
    |     out=[t+48,o+48];
    | end
  function out=numberText3(in):
    | function out=numberText3(in)
    | % This function takes a number (in) and converts it to
    | % a three-digit character output. Useful for VCODES.
    |     o=floor(mod(in,10));
    |     t=floor(mod(in,100)/10);
    |     h=floor(in/100);
    | 
    |     out=[h+48,t+48,o+48];
    | end

== matlab function Embedded MATLAB Function2 ==
  data: perturb input double; Fout output double
function Fout = loads(perturb)

    persistent force ramp;
    
    if isempty(ramp)
        ramp=zeros(150,1);
        ramp(1:50)=1:50;
        ramp(51:100)=50;
        ramp(101:150)=50:-1:1;
        ramp=ramp/max(ramp);
    end
    
    if isempty(force)
        force=zeros(150,4);
    end
    
    force=force+ramp*perturb;
    
    force(1:149,:)=force(2:150,:);force(end,:)=0;
    
    Fout=force(1,:);
    
end

== matlab function Process_Video_CMD/EML ==
  settings: fimath=|
      | fimath(...
      | 'RoundMode', 'floor',...
      | 'OverflowMode', 'wrap',...
      | 'ProductMode', 'KeepLSB', 'ProductWordLength', 32,...
      | 'SumMode', 'KeepLSB', 'SumWordLength', 32,...
      | 'CastBeforeSum', false)
  data: USER_VCODES input double; VCODEs_out output double; GUI_VCODES input double; num_used_VCODEs output double
function [VCODEs_out,num_used_VCODEs] = fcn(USER_VCODES, GUI_VCODES)

% set the maximum number of user VCODEs allowed (although the actual number displayed may be cropped by the UDP packet size)
max_num_USER_VCODES = 80;			

num_USER_VCODEs = size(USER_VCODES, 1);
num_GUI_VCODEs = size(GUI_VCODES, 1);

USER_VCODE_length = size(USER_VCODES, 2);
GUI_VCODE_length = size(GUI_VCODES, 2);

if USER_VCODE_length == 1
	% this situation will happen if there are no USER_VCODEs
	VCODEs_out = [GUI_VCODES; zeros(max_num_USER_VCODES, GUI_VCODE_length)];
	num_USER_VCODEs = 0;
elseif	num_USER_VCODEs > max_num_USER_VCODES
	% limit the number of user VCODEs to ensure that the total number does not exceed the max_num_USER_VCODES
	VCODEs_out = [USER_VCODES(1:max_num_USER_VCODES, :); GUI_VCODES];
	num_USER_VCODEs = max_num_USER_VCODES;
else
	% use all of the USER_VCODEs
	VCODEs_out = [USER_VCODES; GUI_VCODES; zeros(max_num_USER_VCODES - num_USER_VCODEs, USER_VCODE_length)];
end

num_used_VCODEs = num_USER_VCODEs + num_GUI_VCODEs;
